simulink model "Single_Phase_Vienna_Rectifier_DPWM"  (R2021b)
settings: Solver=VariableStepAuto  StartTime=0.0  StopTime=2  RelTol=1e-3
libraries: spsMeanLib x4, spsDiodeLib x4, spsIGBTDiodeLib x4, spsVoltageMeasurementLib x4, simulink x4, spsCurrentMeasurementLib x3, spsSeriesRLCBranchLib x3, spsACVoltageSourceLib x1, spsMutualInductanceLib x1, slpidlib x1, powerlib_extras x1, spsTHDLib x1
settings Model: SimulationMode=accelerator  Creator=abc6820292  LastModifiedBy=abc6820292

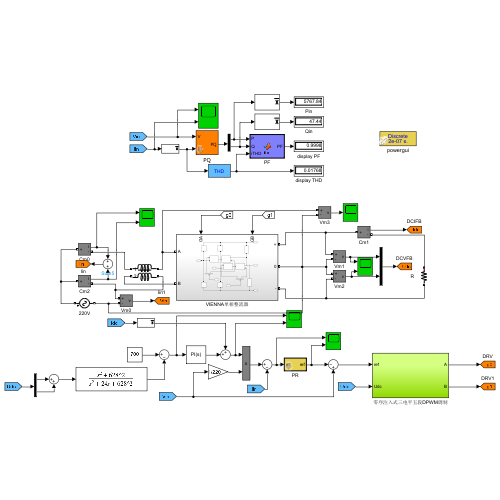
[thumbnail: Simulink's stored preview of the top-level diagram]
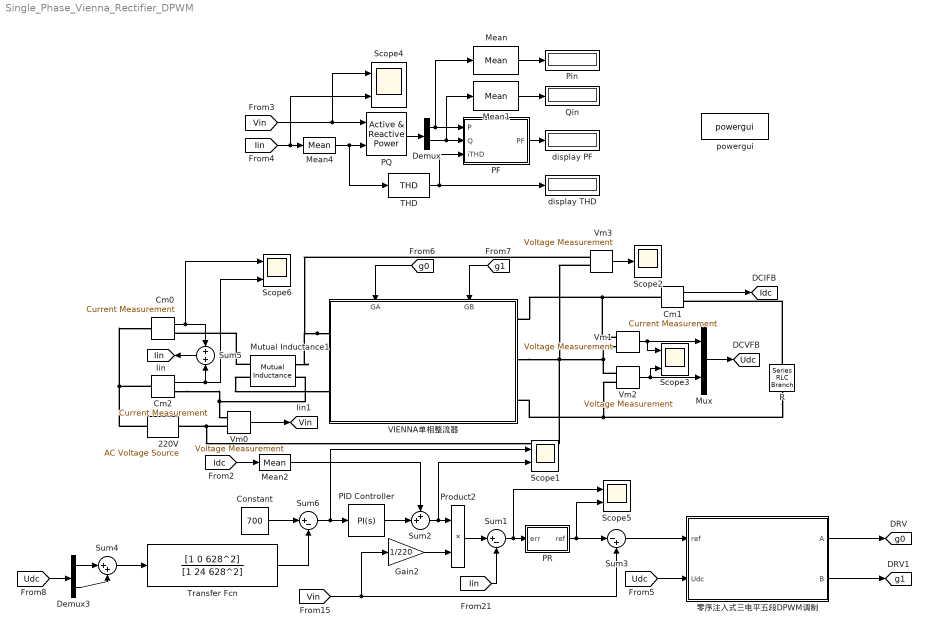
== system Single_Phase_Vienna_Rectifier_DPWM ==
  220V : spsACVoltageSourceLib/AC Voltage Source  Amplitude=311  Phase=0  Frequency=50  SampleTime=0  Measurements=None  BusType=swing  Pref=10e3  Qref=0  Qmin=-inf  Qmax=+inf
  Cm0 : spsCurrentMeasurementLib/Current Measurement  PhasorSimulation=off  OutputType=Complex  PSBequivalent=0
  Cm1 : spsCurrentMeasurementLib/Current Measurement  PhasorSimulation=off  OutputType=Complex  PSBequivalent=0
  Cm2 : spsCurrentMeasurementLib/Current Measurement  PhasorSimulation=off  OutputType=Complex  PSBequivalent=0
  Constant : Constant  Value=700
  Demux : Demux  Outputs=2
  Demux3 : Demux  Outputs=2
  Gain2 : Gain  Gain=1/220
  Mean : spsMeanLib/Mean  Freq=50  Vinit=0  Ts=0
  Mean1 : spsMeanLib/Mean  Freq=50  Vinit=0  Ts=0
  Mean2 : spsMeanLib/Mean  Freq=50  Vinit=0  Ts=0
  Mean4 : spsMeanLib/Mean  Freq=16000  Vinit=0  Ts=0
  Mutual Inductance1 : spsMutualInductanceLib/Mutual Inductance  LConnTagsString=a|b  RConnTagsString=A|B  TypeOfMutual=Two or three windings with equal mutual terms  NumberOfWindings=3  SelfImpedance1=[0.01 1.5e-3]  SelfImpedance2=[0.01 1.5e-3]  ThreeWindings=off  SelfImpedance3=[ 1.1 1.1e-03]  MutualImpedance=[0.02 1e-3]  InductanceMatrix="[1.0 0.9  0.9 ;  0.9 1.0  0.9;  0.9 0.9 1.0 ] * 1e-3"  ResistanceMatrix="[1.0 0.9  0.9 ;  0.9 1.0  0.9;  0.9 0.9 1.0 ]"  Measurements=None
      settings: SourceProductBaseCode=PS
  Mux : Mux  Inputs=2
  PF : MATLAB Function  TreatAsAtomicUnit=on
  PID Controller : slpidlib/PID Controller  Controller=PI  Form=Parallel  TimeDomain=Continuous-time  UseExternalTs=off  SampleTime=-1  IntegratorMethod=Forward Euler  FilterMethod=Forward Euler  ControllerParametersSource=internal  P=0.1  I=2  D=0.005  UseFilter=on  N=100  TunerSelectOption=Transfer Function Based (PID Tuner App)  InitialConditionSource=internal  InitialConditionForIntegrator=0  InitialConditionForFilter=0  DifferentiatorICPrevScaledInput=0  ExternalReset=none  TrackingMode=off  Kt=1  LimitOutput=off  SatLimitsSource=internal  UpperSaturationLimit=200  LowerSaturationLimit=0  LinearizeAsGain=on  AntiWindupMode=clamping  Kb=1  POutMin=[]  POutMax=[]  IOutMin=[]  IOutMax=[]  DOutMin=[]  DOutMax=[]  NOutMin=[]  NOutMax=[]  SumOutMin=[]  SumOutMax=[]  SaturationOutMin=[]  SaturationOutMax=[]  PParamMin=[]  PParamMax=[]  IParamMin=[]  IParamMax=[]  DParamMin=[]  DParamMax=[]  NParamMin=[]  NParamMax=[]  KbParamMin=[]  KbParamMax=[]  KtParamMin=[]  KtParamMax=[]  KbOutMin=[]  KbOutMax=[]  KtOutMin=[]  KtOutMax=[]  IntegratorOutMin=[]  IntegratorOutMax=[]  FilterOutMin=[]  FilterOutMax=[]  SumI1OutMin=[]  SumI1OutMax=[]  SumI2OutMin=[]  SumI2OutMax=[]  SumI3OutMin=[]  SumI3OutMax=[]  SumI4OutMin=[]  SumI4OutMax=[]  SumDOutMin=[]  SumDOutMax=[]  DifferentiatorOutMin=[]  DifferentiatorOutMax=[]  FilterDiffOutCoefMin=[]  FilterDiffOutCoefMax=[]  ReciprocalOutMin=[]  ReciprocalOutMax=[]  SumDenOutMin=[]  SumDenOutMax=[]  SumNumOutMin=[]  SumNumOutMax=[]  DivideOutMin=[]  DivideOutMax=[]  UdiffTsProdOutMin=[]  UdiffTsProdOutMax=[]  NTsProdOutMin=[]  NTsProdOutMax=[]  UintegralTsProdOutMin=[]  UintegralTsProdOutMax=[]  UngainTsProdOutMin=[]  UngainTsProdOutMax=[]  FilterDenConstantOutDataTypeStr=Inherit: Inherit via back propagation  FilterDenConstantOutMin=[]  FilterDenConstantOutMax=[]  PCopyOutDataTypeStr=Inherit: Inherit via back propagation  PCopyOutMin=[]  PCopyOutMax=[]  NCopyOutDataTypeStr=Inherit: Inherit via back propagation  NCopyOutMin=[]  NCopyOutMax=[]  IntegratorContinuousStateAttributes=''  IntegratorStateMustResolveToSignalObject=off  IntegratorRTWStateStorageClass=Auto  FilterContinuousStateAttributes=''  FilterStateMustResolveToSignalObject=off  FilterRTWStateStorageClass=Auto  ParallelPVariant=InternalParameters  IdealPVariant=Disabled  IVariant=InternalParameters  DVariant=Disabled  IntegratorVariant=Continuous  SatVariant=Disabled  AWVariant=Passthrough  PCopyVariant=Disabled  TRVariant=Disabled  FdbkBlocksVariant=Forward  IdealPFdbkVariant=Disabled  SatFdbkVariant=Disabled  DerivativeFilterVariant=Disabled  NVariant=Disabled  NCopyVariant=Disabled_SignalSpec  FilterICVariant=Disabled  IntegratorICVariant=InternalICs  ExternalResetVariant=Disabled  TRSumVariant=Passthrough  SumFdbkVariant=Disabled  SumVariant=Sum_PI  TsampFilterVariant=InternalTs  TsampNgainVariant=Passthrough  TsampIntegralVariant=Passthrough  ExternalSaturationOutDataTypeStr=Inherit: Same as second input
  PQ : powerlib_extras/Measurements/Active & Reactive Power  f1=50
      settings: SourceProductBaseCode=PS
  PR : Subsystem  TreatAsAtomicUnit=on  mask{Kp=3, Kr=50, Wc=5, Upper=100, Lower=-100}
  Pin : Display
      settings: Format=bank
  Product2 : Product  RndMeth=Zero
  Qin : Display
      settings: Format=bank
  R : spsSeriesRLCBranchLib/Series RLC Branch  LConnTagsString=__new0  RConnTagsString=__new0  BranchType=R  Resistance=100  Inductance=7e-4  SetiL0=off  InitialCurrent=0  Capacitance=1e-3  Setx0=off  InitialVoltage=0  Measurements=None
  Scope{1,3..6} (5 alike) : Scope  NumInputPorts=2
  Scope2 : Scope
  Sum1 : Sum  Inputs=|+-
  Sum2 : Sum  Inputs=++|
  Sum3 : Sum  Inputs=|-+
  Sum4 : Sum  Inputs=|++
  Sum5 : Sum  Inputs=+|+
  Sum6 : Sum  Inputs=|+-
  THD : spsTHDLib/THD  Freq=50  Ts=0
      settings: SourceProductBaseCode=PS
  Transfer Fcn : TransferFcn  Numerator=[1 0 628^2]  Denominator=[1 24 628^2]
  VIENNA单相整流器 : Subsystem
      settings: PortSchema="{\"entries\":[{\"content\":{\"sides\":[{\"content\":{\"connectorIds\":[\"LConn1\",\"LConn2\",\"LConn3\"]},\"type\":\"ConnectorPlacement.EquallySpacedRectSide\",\"uuid\":\"47187a24-6853-42ac-9ad9-0df0e1360fae\"},{\"content\":{\"connectorIds\":[\"RConn1\",\"RConn2\"],\"side\":\"RIGHT\"},\"type\":\"ConnectorPlacement.EquallySpacedRectSide\",\"uuid\":\"b3504369-b235-4116-9b9b-167bd6b76527\"},{\"content\":{\"connectorIds\":[\"In1\",\"In2\"],\"side\":\"TOP\"},\"type\":\"ConnectorPlacement.EquallySpacedRectSide\",\"uuid\":\"5cb205b4-da18-4f20-b3d4-22846a9c2236\"},{\"content\":{\"connectorIds\":[],\"side\":\"BOTTOM\"},\"type\":\"ConnectorPlacement.EquallySpacedRectSide\",\"uuid\":\"4e548a82-6bdf-470e-8572-00c7c8855d01\"}]},\"type\":\"ConnectorPlacement.EquallySpacedConnector\",\"uuid\":\"b00ba750-ea4b-4b64-a122-5cbc9e899126\"}],\"packageUris\":[\"http://schema.mathworks.com/mf0/Connector/R2020b\"],\"version\":\"1.0\"}"
  Vm{0..3} (4 alike) : spsVoltageMeasurementLib/Voltage Measurement  PhasorSimulation=off  OutputType=Complex  PSBequivalent=0
  display PF : Display
  display THD : Display
  powergui : spspowerguiLib/powergui  SimulationMode=Discrete  SampleTime=2e-7  frequency=60  Iterations=50  frequencyindice=0  Pbase=100e6  ErrMax=1e-4  UnitsV=kV  UnitsW=MW  buscounter=0  FunctionMessages=off  echomessages=off  EnableUseOfTLC=off  CurrentSourceSwitches=off  DisableSnubberDevices=off  DisableRonSwitches=off  DisableVfSwitches=off  DisplayEquations=off  AutomaticDiscreteSolvers=off  SolverType=Tustin/Backward Euler (TBE)  Interpol=off  ExternalGateDelay=off  methode=off  Ts=0  x0status=blocks  SPID=off  SwTol=0  HookPort=off  NonlinearTolerance=1e-4  nMaxIteration=100  ContinueOnMaxIteration=off  RestoreLinks=warning  ResistiveCurrentMeasurement=off  Frange=[0:2:500]  Ylog=off  Xlog=on  ShowGrid=off  save=off  variable=ZData  structure=QQQQQ  ZoomFFT=off  StartTime=0.5  cycles=15  DisplayStyle=1  fundamental=50  FreqAxis=off  MaxFrequency=1000  frequencyindicesteady=1  RmsSteady=1  display=off
  零序注入式三电平五段DPWM调制 : Subsystem
  tag scope: Idc=global, Iin=global, Udc=global, Vin=global, g0=global, g1=global
  wires:
  Demux3/1 -> Sum4/1
  [Vin] -> Gain2/1, Sum3/2
  PQ/1 -> Demux/1
  Transfer Fcn/1 -> Sum6/2
  Sum2/1 -> Scope1/2, Product2/1
  Mux/1 -> [Udc]
  Mean4/1 -> THD/1, PQ/2
  THD/1 -> display THD/1, PF/3(iTHD)
  Sum4/1 -> Transfer Fcn/1
  [Iin] -> Scope4/2, Mean4/1
  [g0] -> VIENNA单相整流器/2(GA)
  PID Controller/1 -> Sum2/2
  Demux/2 -> Mean1/1, PF/2(Q)
  Product2/1 -> Sum1/1
  零序注入式三电平五段DPWM调制/1(A) -> [g0]
  Vm1/1 -> Scope3/1, Mux/1
  [Udc] -> Demux3/1
  Sum1/1 -> Scope5/1, PR/1(err)
  Sum3/1 -> 零序注入式三电平五段DPWM调制/1(ref)
  [Iin] -> Sum1/2
  Vm0/1 -> [Vin]
  Sum6/1 -> PID Controller/1, Scope1/1
  Gain2/1 -> Product2/2
  [Idc] -> Mean2/1
  [Vin] -> Scope4/1, PQ/1
  零序注入式三电平五段DPWM调制/2(B) -> [g1]
  Mean2/1 -> Sum2/1
  Mean/1 -> Pin/1
  PF/1(PF) -> display PF/1
  Demux3/2 -> Sum4/2
  [Udc] -> 零序注入式三电平五段DPWM调制/2(Udc)
  [g1] -> VIENNA单相整流器/1(GB)
  Demux/1 -> Mean/1, PF/1(P)
  Vm2/1 -> Scope3/2, Mux/2
  Cm1/1 -> [Idc]
  Mean1/1 -> Qin/1
  PR/1(ref) -> Sum3/1, Scope5/2
  Constant/1 -> Sum6/1
  Cm0/1 -> Scope6/1, Sum5/1
  Cm2/1 -> Scope6/2, Sum5/2
  Sum5/1 -> [Iin]
  Vm3/1 -> Scope2/1
  connections:
  R/RConn1 -- Vm2/LConn2 -- VIENNA单相整流器/LConn3
  Mutual Inductance1/LConn1 -- Cm0/RConn1
  Cm1/LConn1 -- Vm1/LConn1 -- VIENNA单相整流器/LConn1
  Vm0/LConn2 -- Vm3/LConn2 -- Vm2/LConn1 -- Vm1/LConn2 -- VIENNA单相整流器/LConn2 -- 220V/LConn1
  R/LConn1 -- Cm1/RConn1
  220V/RConn1 -- Cm2/LConn1 -- Cm0/LConn1
  VIENNA单相整流器/RConn1 -- Mutual Inductance1/RConn1 -- Vm3/LConn1
  Cm2/RConn1 -- Vm0/LConn1 -- Mutual Inductance1/RConn2
  Mutual Inductance1/LConn2 -- VIENNA单相整流器/RConn2

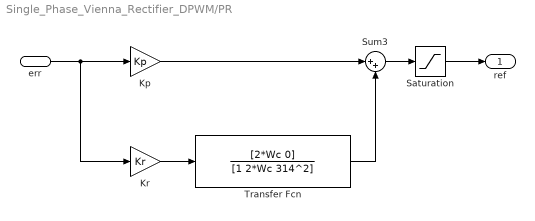
== system Single_Phase_Vienna_Rectifier_DPWM/PR ==
  err : Inport
  Kp : Gain  Gain=Kp
  Kr : Gain  Gain=Kr
  Saturation : Saturate  UpperLimit=Upper  LowerLimit=Lower
  Sum3 : Sum  Inputs=|++
  Transfer Fcn : TransferFcn  Numerator=[2*Wc 0]  Denominator=[1 2*Wc 314^2]
  ref : Outport
  wires:
  Kp/1 -> Sum3/1
  Sum3/1 -> Saturation/1
  err/1 -> Kr/1, Kp/1
  Kr/1 -> Transfer Fcn/1
  Transfer Fcn/1 -> Sum3/2
  Saturation/1 -> ref/1

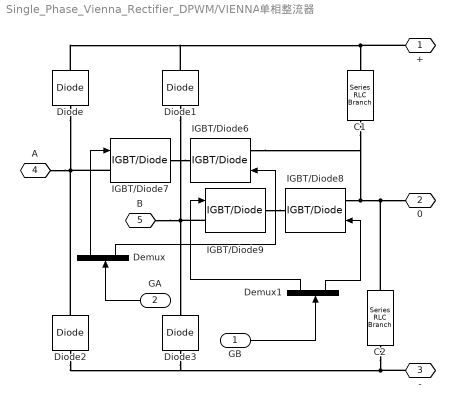
== system Single_Phase_Vienna_Rectifier_DPWM/VIENNA单相整流器 ==
  GB : Inport
  GA : Inport  Port=2
  C1 : spsSeriesRLCBranchLib/Series RLC Branch  LConnTagsString=__new0  RConnTagsString=__new0  BranchType=C  Resistance=0  Inductance=0  SetiL0=off  InitialCurrent=0  Capacitance=4e-3  Setx0=on  InitialVoltage=310  Measurements=None
  C2 : spsSeriesRLCBranchLib/Series RLC Branch  LConnTagsString=__new0  RConnTagsString=__new0  BranchType=C  Resistance=0.1  Inductance=0  SetiL0=off  InitialCurrent=0  Capacitance=4e-3  Setx0=on  InitialVoltage=310  Measurements=None
  Demux : Demux  Outputs=2
  Demux1 : Demux  Outputs=2
  Diode{,1..3} (4 alike) : spsDiodeLib/Diode  Ron=0.001  Lon=0  Vf=0.8  IC=0  UseSnubber=0  Rs=5e6  Cs=25e-9  Measurements=off
  IGBT/Diode{6..9} (4 alike) : spsIGBTDiodeLib/IGBT//Diode  Ron=1e-3  Rs=1e5  Cs=inf  Measurements=off
  + : PMIOPort  Side=Left
  0 : PMIOPort  Port=2  Side=Left
  - : PMIOPort  Port=3  Side=Left
  A : PMIOPort  Port=4  Side=Right
  B : PMIOPort  Port=5  Side=Right
  wires:
  GA/1 -> Demux/1
  GB/1 -> Demux1/1
  Demux/2 -> IGBT/Diode6/1
  Demux/1 -> IGBT/Diode7/1
  Demux1/2 -> IGBT/Diode8/1
  Demux1/1 -> IGBT/Diode9/1
  connections:
  IGBT/Diode9/LConn1 -- Diode3/RConn1 -- Diode1/LConn1 -- B/RConn1
  +/RConn1 -- Diode1/RConn1 -- Diode/RConn1 -- C1/LConn1
  -/RConn1 -- Diode2/LConn1 -- Diode3/LConn1 -- C2/RConn1
  A/RConn1 -- Diode2/RConn1 -- Diode/LConn1 -- IGBT/Diode7/LConn1
  IGBT/Diode7/RConn1 -- IGBT/Diode6/RConn1
  IGBT/Diode8/LConn1 -- C1/RConn1 -- IGBT/Diode6/LConn1 -- C2/LConn1 -- 0/RConn1
  IGBT/Diode9/RConn1 -- IGBT/Diode8/RConn1

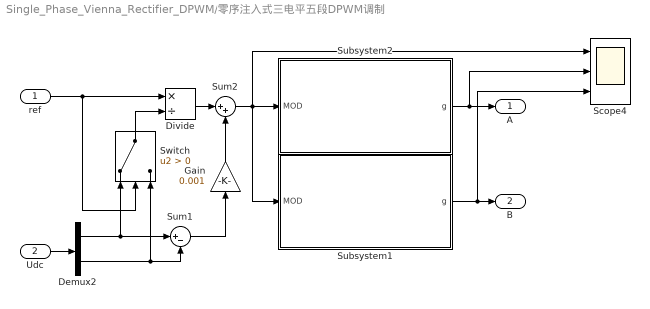
== system Single_Phase_Vienna_Rectifier_DPWM/零序注入式三电平五段DPWM调制 ==
  ref : Inport
  Udc : Inport  Port=2
  Demux2 : Demux  Outputs=2
  Divide : Product  Inputs=*/
  Gain : Gain  Gain=0.001
  Scope4 : Scope  NumInputPorts=3
  Subsystem1 : Subsystem
  Subsystem2 : Subsystem
  Sum1 : Sum  Inputs=|+-
  Sum2 : Sum  Inputs=|++
  Switch : Switch  Criteria=u2 > Threshold
  A : Outport
  B : Outport  Port=2
  wires:
  Subsystem2/1(g) -> Scope4/2, A/1
  Udc/1 -> Demux2/1
  Sum1/1 -> Gain/1
  Sum2/1 -> Subsystem1/1(MOD), Scope4/1, Subsystem2/1(MOD)
  Divide/1 -> Sum2/1
  ref/1 -> Divide/1, Switch/2
  Switch/1 -> Divide/2
  Demux2/1 -> Sum1/1, Switch/1
  Demux2/2 -> Sum1/2, Switch/3
  Gain/1 -> Sum2/2
  Subsystem1/1(g) -> Scope4/3, B/1

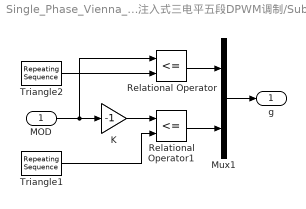
== system Single_Phase_Vienna_Rectifier_DPWM/零序注入式三电平五段DPWM调制/Subsystem1 ==
  MOD : Inport
  K : Gain  Gain=-1
  Mux1 : Mux  Inputs=2
  Relational Operator : RelationalOperator  Operator=<=  OutDataTypeStr=boolean  RndMeth=Nearest
  Relational Operator1 : RelationalOperator  Operator=<=  OutDataTypeStr=boolean  RndMeth=Nearest
  Triangle1 : simulink/Sources/Repeating Sequence  rep_seq_t=[0 1/40000/2 1/40000]  rep_seq_y=[0 1 0]
  Triangle2 : simulink/Sources/Repeating Sequence  rep_seq_t=[0 1/40000/2 1/40000]  rep_seq_y=[1 0 1]
  g : Outport
  wires:
  MOD/1 -> Relational Operator/1, K/1
  Mux1/1 -> g/1
  K/1 -> Relational Operator1/1
  Relational Operator/1 -> Mux1/1
  Relational Operator1/1 -> Mux1/2
  Triangle2/1 -> Relational Operator/2
  Triangle1/1 -> Relational Operator1/2

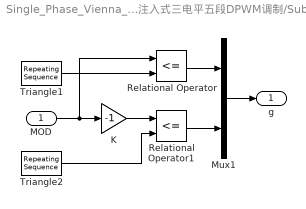
== system Single_Phase_Vienna_Rectifier_DPWM/零序注入式三电平五段DPWM调制/Subsystem2 ==
  MOD : Inport
  K : Gain  Gain=-1
  Mux1 : Mux  Inputs=2
  Relational Operator : RelationalOperator  Operator=<=  OutDataTypeStr=boolean  RndMeth=Nearest
  Relational Operator1 : RelationalOperator  Operator=<=  OutDataTypeStr=boolean  RndMeth=Nearest
  Triangle1 : simulink/Sources/Repeating Sequence  rep_seq_t=[0 1/40000/2 1/40000]  rep_seq_y=[0 1 0]
  Triangle2 : simulink/Sources/Repeating Sequence  rep_seq_t=[0 1/40000/2 1/40000]  rep_seq_y=[1 0 1]
  g : Outport
  wires:
  MOD/1 -> Relational Operator/1, K/1
  Triangle1/1 -> Relational Operator/2
  Mux1/1 -> g/1
  K/1 -> Relational Operator1/1
  Triangle2/1 -> Relational Operator1/2
  Relational Operator/1 -> Mux1/1
  Relational Operator1/1 -> Mux1/2

== matlab function Single_Phase_Vienna_Rectifier_DPWM/PF ==
  data: P input; PF output; Q input; iTHD input
function PF = fcn(P,Q,iTHD)
% This block supports an embeddable subset of the MATLAB language.
% See the help menu for details. 
PF=(P/sqrt(P*P+Q*Q))/(sqrt(1+iTHD*iTHD));
